simulink model "gm_PMLSM_FOC_FixedPoint"  (R2026b)
settings: Solver=FixedStepDiscrete  StopTime=0.0063  FixedStep=2e-08
undefined symbols (not defined in the file): Lookup, Ts_ACR
libraries: hdlmdlgenlib x38, simulink x8
(part 2 of 5)

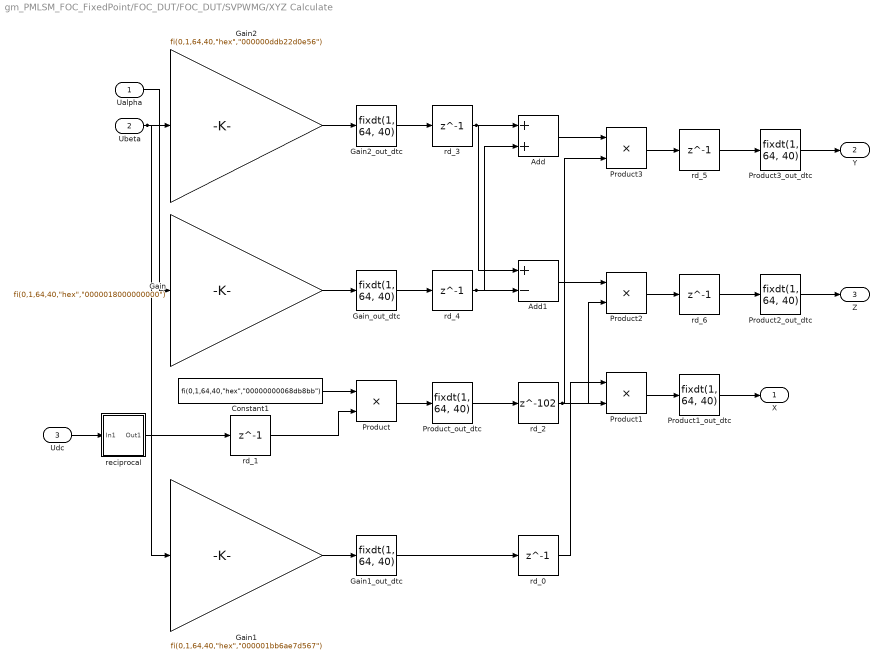
== system gm_PMLSM_FOC_FixedPoint/FOC_DUT/FOC_DUT/SVPWMG/XYZ Calculate ==
  Ualpha : Inport  OutDataTypeStr=fixdt(1, 64, 40)  PortDimensions=1  SampleTime=2e-08
  Ubeta : Inport  Port=2  OutDataTypeStr=fixdt(1, 64, 40)  PortDimensions=1  SampleTime=2e-08
  Udc : Inport  Port=3  OutDataTypeStr=fixdt(0, 32, 24)  PortDimensions=1  SampleTime=2e-08
  Add : Sum  OutDataTypeStr=fixdt(1, 64, 40)  AccumDataTypeStr=fixdt(1, 64, 40)  RndMeth=Convergent  SaturateOnIntegerOverflow=on  SampleTime=2e-08
  Add1 : Sum  Inputs=+-  OutDataTypeStr=fixdt(1, 64, 40)  AccumDataTypeStr=fixdt(1, 64, 40)  RndMeth=Convergent  SaturateOnIntegerOverflow=on  SampleTime=2e-08
  Constant1 : Constant  Value="fi(0,1,64,40,\"hex\",\"00000000068db8bb\")"  OutDataTypeStr=fixdt(1, 64, 40)  SampleTime=2e-08
  Gain : Gain  Gain="fi(0,1,64,40,\"hex\",\"0000018000000000\")"  ParamDataTypeStr=fixdt(1, 64, 40)  OutDataTypeStr=fixdt(1, 128, 80)  SampleTime=2e-08
  Gain1 : Gain  Gain="fi(0,1,64,40,\"hex\",\"000001bb6ae7d567\")"  ParamDataTypeStr=fixdt(1, 64, 40)  OutDataTypeStr=fixdt(1, 128, 80)  SampleTime=2e-08
  Gain1_out_dtc : DataTypeConversion  OutDataTypeStr=fixdt(1, 64, 40)  RndMeth=Convergent  SampleTime=2e-08
  Gain2 : Gain  Gain="fi(0,1,64,40,\"hex\",\"000000ddb22d0e56\")"  ParamDataTypeStr=fixdt(1, 64, 40)  OutDataTypeStr=fixdt(1, 128, 80)  SampleTime=2e-08
  Gain2_out_dtc : DataTypeConversion  OutDataTypeStr=fixdt(1, 64, 40)  RndMeth=Convergent  SampleTime=2e-08
  Gain_out_dtc : DataTypeConversion  OutDataTypeStr=fixdt(1, 64, 40)  RndMeth=Convergent  SampleTime=2e-08
  Product{,1..3} (4 alike) : Product  Inputs=**  OutDataTypeStr=fixdt(1, 128, 80)  SampleTime=2e-08
  Product1_out_dtc : DataTypeConversion  OutDataTypeStr=fixdt(1, 64, 40)  RndMeth=Convergent  SampleTime=2e-08
  Product2_out_dtc : DataTypeConversion  OutDataTypeStr=fixdt(1, 64, 40)  RndMeth=Convergent  SampleTime=2e-08
  Product3_out_dtc : DataTypeConversion  OutDataTypeStr=fixdt(1, 64, 40)  RndMeth=Convergent  SampleTime=2e-08
  Product_out_dtc : DataTypeConversion  OutDataTypeStr=fixdt(1, 64, 40)  RndMeth=Convergent  SampleTime=2e-08
  rd_{0..1,3..6} (6 alike) : Delay  DelayLength=1  InitialCondition=0  SampleTime=2e-08
  rd_2 : Delay  DelayLength=102  InitialCondition=0  SampleTime=2e-08
  reciprocal : Subsystem
  X : Outport  OutDataTypeStr=fixdt(1, 64, 40)  PortDimensions=1  SampleTime=2e-08
  Y : Outport  Port=2  OutDataTypeStr=fixdt(1, 64, 40)  PortDimensions=1  SampleTime=2e-08
  Z : Outport  Port=3  OutDataTypeStr=fixdt(1, 64, 40)  PortDimensions=1  SampleTime=2e-08
  wires:
  rd_3/1 -> Add1/1, Add/1
  Udc/1 -> reciprocal/1(In1)
  Ualpha/1 -> Gain/1
  Ubeta/1 -> Gain2/1, Gain1/1
  Gain2/1 -> Gain2_out_dtc/1
  Gain1_out_dtc/1 -> rd_0/1
  reciprocal/1(Out1) -> rd_1/1
  rd_1/1 -> Product/2
  Gain/1 -> Gain_out_dtc/1
  Constant1/1 -> Product/1
  Gain1/1 -> Gain1_out_dtc/1
  Gain2_out_dtc/1 -> rd_3/1
  Gain_out_dtc/1 -> rd_4/1
  Product/1 -> Product_out_dtc/1
  rd_4/1 -> Add1/2, Add/2
  Product_out_dtc/1 -> rd_2/1
  Add/1 -> Product3/1
  Product1/1 -> Product1_out_dtc/1
  Add1/1 -> Product2/1
  rd_2/1 -> Product1/2, Product3/2, Product2/2
  rd_0/1 -> Product1/1
  Product3/1 -> rd_5/1
  Product2/1 -> rd_6/1
  rd_5/1 -> Product3_out_dtc/1
  Product1_out_dtc/1 -> X/1
  rd_6/1 -> Product2_out_dtc/1
  Product3_out_dtc/1 -> Y/1
  Product2_out_dtc/1 -> Z/1

== system gm_PMLSM_FOC_FixedPoint/FOC_DUT/FOC_DUT/dq_voltage_limiter/Divide ==
  In1 : Inport
  In2 : Inport  Port=2
  Divide : Product  Inputs=*/  OutDataTypeStr=FOC_Fixed_Config.Types.DivideWide  RndMeth=Convergent  SaturateOnIntegerOverflow=on
  Divide_pd1 : Delay  DelayLength=109
  Out1 : Outport
  wires:
  Divide_pd1/1 -> Out1/1
  In1/1 -> Divide/1
  In2/1 -> Divide/2
  Divide/1 -> Divide_pd1/1

== system gm_PMLSM_FOC_FixedPoint/FOC_DUT/FOC_DUT/dq_voltage_limiter/Sqrt ==
  In1 : Inport
  Delay2 : Delay  DelayLength=56
  Sqrt : Sqrt  OutDataTypeStr=FOC_Fixed_Config.Types.Work
  Out1 : Outport
  wires:
  In1/1 -> Sqrt/1
  Sqrt/1 -> Delay2/1
  Delay2/1 -> Out1/1

== system gm_PMLSM_FOC_FixedPoint/FOC_DUT/FOC_DUT/InversePark/Variant/mcb ==
  A : Inport  OutDataTypeStr=fixdt(1, 64, 40)  PortDimensions=1  SampleTime=2e-08
  B : Inport  Port=2  OutDataTypeStr=fixdt(1, 64, 40)  PortDimensions=1  SampleTime=2e-08
  C : Inport  Port=3  OutDataTypeStr=fixdt(1, 40, 32)  PortDimensions=1  SampleTime=0.0001
  Inverse Park Transform : Subsystem  mask(Inverse Park Transform){PhaseInput=Two inputs, AxisAlignment=D-axis, ThetaInput=Sine and Cosine electrical position, AngleInput=Per-unit, N_points=1024}
      mask prompts: PhaseInput "mcb:CtrlLib:InvPPrmInp"; AxisAlignment "mcb:CtrlLib:InvPBlkPrmAlign"; ThetaInput "mcb:CtrlLib:InvPPrmTheta"; AngleInput "shared_mcbeeblks:mcbeeblks:InvPThetaUnits"; N_points "mcb:CtrlLib:SineBlkPrmLUTSize"
      mask help: mcb:CtrlLib:InvPBlkDlgDes
      mask init:
      | AngleInput = 2;
      | AxisAlignment = 'D-axis';
      | N_points = 1024;
      | PhaseInput = 1;
      | ThetaInput = 1;
      | dlgSett = struct('Offset', 0);
      mask Help: eval('mcb_helpview(''inverseparktransform'')')
      mask TypeOptions PhaseInput: shared_mcbeeblks:mcbeeblks:InvPPopTwo | shared_mcbeeblks:mcbeeblks:InvPPopThree
      mask TypeOptions AxisAlignment: D-axis | Q-axis
      mask TypeOptions ThetaInput: shared_mcbeeblks:mcbeeblks:InvPPopSinCos
      mask TypeOptions AngleInput: shared_mcbeeblks:mcbeeblks:InvPPopRadUnit | shared_mcbeeblks:mcbeeblks:InvPPopPUUnit | shared_mcbeeblks:mcbeeblks:InvPPopDegUnit
      mask Display:
      | port_label('input', 1, 'd', 'texmode', 'on');
      | port_label('input', 2, 'q', 'texmode', 'on');
      | port_label('input', 3, 'sin\theta_e', 'texmode', 'on');
      | port_label('input', 4, 'cos\theta_e', 'texmode', 'on');
      | port_label('output', 1, '\alpha', 'texmode', 'on');
      | port_label('output', 2, '\beta', 'texmode', 'on');
      | fprintf('Inverse Park\nTransform')
  sinecos : Subsystem  mask(SinCos Embedded Optimized){OptforProc=off, OptLevelPop=Disabled, ApproximationMethod='None', UserApproxMethod=Lookup, ApproxStatus=Lookup, ThetaDataType=single, CopyThetaDataType=single, InterpMethod='Linear point-slope', NumberOfDataPoints=16, NumberOfIterations=11, RemoveProtectionAgainstOutOfRangeInput='off', TableDataTypeStr='Inherit: Inherit via input', AngleInput='Radians', CopyAngleInput=Radians, N_points=N_points, CopyN_points=1024, Datatype='Inherit: Same as input', CopyTableDatatype=Inherit: Same as input, DatatypeInput='Inherit from input', IsPrevStrictOpt=0, IsPrevLUTForced=0}
      mask prompts: OptforProc "shared_mcbpccmath:SinCosLib:SineBlkOptimizeChkBox"; OptLevelPop "shared_mcbpccmath:SinCosLib:SineBlkOptimizePopMenu"; ApproximationMethod "Simulink:blkprm_prompts:ApproximationMethod"; UserApproxMethod "Simulink:blkprm_prompts:ApproximationMethod"; ApproxStatus "Simulink:blkprm_prompts:ApproximationMethod"; ThetaDataType "shared_mcbpccmath:SinCosLib:SineBlkPrmThetatype"; CopyThetaDataType "shared_mcbpccmath:SinCosLib:SineBlkPrmThetatype"; InterpMethod "Simulink:blkprm_prompts:InterpndInterpMethod"; NumberOfDataPoints "SimulinkBlocks:dialog:NumberOfDataPoints"; NumberOfIterations "SimulinkBlocks:dialog:NumberOfIterations"; RemoveProtectionAgainstOutOfRangeInput "Simulink:blkprm_prompts:TrigRemoveProtectionAgainstOutOfRangeInput"; TableDataTypeStr "Simulink:blkprm_prompts:TABLE_UNIFIEDDATATYPE"; AngleInput "shared_mcbpccmath:SinCosLib:SineBlkPrmUnits"; CopyAngleInput "shared_mcbpccmath:SinCosLib:SineBlkPrmUnits"; N_points "shared_mcbpccmath:SinCosLib:SineBlkPrmLUTSize"; CopyN_points "shared_mcbpccmath:SinCosLib:SineBlkPrmLUTSize"; Datatype "shared_mcbpccmath:SinCosLib:SineBlkPrmDatatype"; CopyTableDatatype "shared_mcbpccmath:SinCosLib:SineBlkPrmDatatype"; DatatypeInput "shared_mcbpccmath:SinCosLib:SineBlkPrmDatatypeInput"; IsPrevStrictOpt "Prev Strict Opt"; IsPrevLUTForced "Prev LUT Forced"
      mask help: mcb:CtrlLib:SineBlkDlgDes
      mask init:
      | AngleInput = 2;
      | ApproxStatus = [];
      | ApproximationMethod = 'None';
      | CopyAngleInput = 2;
      | CopyN_points = 1024;
      | CopyTableDatatype = 'Inherit: Same as input';
      | CopyThetaDataType = 'single';
      | Datatype = 'Inherit: Same as input';
      | DatatypeInput = 1;
      | InterpMethod = 'Linear point-slope';
      | IsPrevLUTForced = 0;
      | IsPrevStrictOpt = 0;
      | N_points = 1024;
      | NumberOfDataPoints = 16;
      | NumberOfIterations = 11;
      | OptLevelPop = 1;
      | OptforProc = 0;
      | RemoveProtectionAgainstOutOfRangeInput = 'off';
      | TableDataTypeStr = 'Inherit: Inherit via input';
      | ThetaDataType = 'single';
      | UserApproxMethod = 2;
      mask Help: eval('mcb_helpview(''sinecosinelookup'')')
      mask TypeOptions OptLevelPop: shared_mcbpccmath:SinCosLib:OptDisablePop | shared_mcbpccmath:SinCosLib:OptThetaOptimizationPop | shared_mcbpccmath:SinCosLib:OptStrictOptimizationPop
      mask Callback OptLevelPop: mcbpccmath.internal.SinCosMaskCb('maskInitFcn',gcbh);
      mask TypeOptions UserApproxMethod: shared_mcbpccmath:SinCosLib:SineApproxNone | shared_mcbpccmath:SinCosLib:SineApproxLookup | shared_mcbpccmath:SinCosLib:SineApproxCORDIC
      mask Callback UserApproxMethod: mcbpccmath.internal.SinCosMaskCb('maskInitFcn',gcbh);
      mask Callback ThetaDataType:
      | mcbpccmath.internal.SinCosMaskCb('updateCopyVar',gcbh,'ThetaDataType');
      | mcbpccmath.internal.SinCosMaskCb('maskInitFcn',gcbh);
      mask Callback AngleInput:
      | mcbpccmath.internal.SinCosMaskCb('updateCopyVar',gcbh,'AngleInput');
      | mcbpccmath.internal.SinCosMaskCb('maskInitFcn',gcbh);
      mask TypeOptions CopyAngleInput: shared_mcbpccmath:SinCosLib:SinePopPUUnit | shared_mcbpccmath:SinCosLib:SinePopRadUnit | shared_mcbpccmath:SinCosLib:SinePopDegUnit
      mask Callback N_points: mcbpccmath.internal.SinCosMaskCb('updateCopyVar',gcbh,'N_points');
      mask Callback Datatype: mcbpccmath.internal.SinCosMaskCb('updateCopyVar',gcbh,'Datatype');
      mask Display: mcbpccmath.internal.drawIcons('Sin-Cos',2);
  O1 : Outport  OutDataTypeStr=fixdt(1, 64, 40)  PortDimensions=1  SampleTime=2e-08
  O2 : Outport  Port=2  OutDataTypeStr=fixdt(1, 64, 40)  PortDimensions=1  SampleTime=2e-08
  wires:
  C/1 -> sinecos/1(Theta)
  A/1 -> Inverse Park Transform/1(Ds)
  Inverse Park Transform/2(Beta) -> O2/1
  B/1 -> Inverse Park Transform/2(Qs)
  sinecos/1(sin) -> Inverse Park Transform/3(Sin)
  sinecos/2(cos) -> Inverse Park Transform/4(Cos)
  Inverse Park Transform/1(Alpha) -> O1/1

== system gm_PMLSM_FOC_FixedPoint/FOC_DUT/FOC_DUT/Park/Variant/mcb ==
  A : Inport  OutDataTypeStr=fixdt(1, 64, 40)  PortDimensions=1  SampleTime=0.0001
  B : Inport  Port=2  OutDataTypeStr=fixdt(1, 64, 40)  PortDimensions=1  SampleTime=0.0001
  C : Inport  Port=3  OutDataTypeStr=fixdt(1, 40, 32)  PortDimensions=1  SampleTime=0.0001
  Park Transform : Subsystem  mask(Park Transform){PhaseInput=Two inputs, AxisAlignment=D-axis, ThetaInput=Sine and Cosine electrical position, AngleInput=Per-unit, N_points=1024}
      mask prompts: PhaseInput "mcb:CtrlLib:ParkPrmInp"; AxisAlignment "mcb:CtrlLib:ParkBlkPrmAlign"; ThetaInput "mcb:CtrlLib:ParkPrmTheta"; AngleInput "shared_mcbeeblks:mcbeeblks:ParkPrmThetaUnits"; N_points "mcb:CtrlLib:SineBlkPrmLUTSize"
      mask help: mcb:CtrlLib:ParkBlkDlgDes
      mask init:
      | AngleInput = 2;
      | AxisAlignment = 'D-axis';
      | N_points = 1024;
      | PhaseInput = 1;
      | ThetaInput = 1;
      | dlgSett = struct('Offset', 0);
      mask Help: eval('mcb_helpview(''parktransform'')')
      mask TypeOptions PhaseInput: shared_mcbeeblks:mcbeeblks:ParkPopTwo | shared_mcbeeblks:mcbeeblks:ParkPopThree
      mask TypeOptions AxisAlignment: D-axis | Q-axis
      mask TypeOptions ThetaInput: shared_mcbeeblks:mcbeeblks:ParkPopSinCos
      mask TypeOptions AngleInput: shared_mcbeeblks:mcbeeblks:ParkPopRadUnit | shared_mcbeeblks:mcbeeblks:ParkPopPUUnit | shared_mcbeeblks:mcbeeblks:ParkPopDegUnit
      mask Display:
      | port_label('input', 1, '\alpha', 'texmode', 'on');
      | port_label('input', 2, '\beta', 'texmode', 'on');
      | port_label('input', 3, 'sin\theta_e', 'texmode', 'on');
      | port_label('input', 4, 'cos\theta_e', 'texmode', 'on');
      | port_label('output', 1, 'd', 'texmode', 'on');
      | port_label('output', 2, 'q', 'texmode', 'on');
      | fprintf('Park\nTransform')
  sinecos : Subsystem  mask(SinCos Embedded Optimized){OptforProc=off, OptLevelPop=Disabled, ApproximationMethod='None', UserApproxMethod=Lookup, ApproxStatus=Lookup, ThetaDataType=single, CopyThetaDataType=single, InterpMethod='Linear point-slope', NumberOfDataPoints=16, NumberOfIterations=11, RemoveProtectionAgainstOutOfRangeInput='off', TableDataTypeStr='Inherit: Inherit via input', AngleInput='Radians', CopyAngleInput=Radians, N_points=N_points, CopyN_points=1024, Datatype='Inherit: Same as input', CopyTableDatatype=Inherit: Same as input, DatatypeInput='Inherit from input', IsPrevStrictOpt=0, IsPrevLUTForced=0}
      mask prompts: OptforProc "shared_mcbpccmath:SinCosLib:SineBlkOptimizeChkBox"; OptLevelPop "shared_mcbpccmath:SinCosLib:SineBlkOptimizePopMenu"; ApproximationMethod "Simulink:blkprm_prompts:ApproximationMethod"; UserApproxMethod "Simulink:blkprm_prompts:ApproximationMethod"; ApproxStatus "Simulink:blkprm_prompts:ApproximationMethod"; ThetaDataType "shared_mcbpccmath:SinCosLib:SineBlkPrmThetatype"; CopyThetaDataType "shared_mcbpccmath:SinCosLib:SineBlkPrmThetatype"; InterpMethod "Simulink:blkprm_prompts:InterpndInterpMethod"; NumberOfDataPoints "SimulinkBlocks:dialog:NumberOfDataPoints"; NumberOfIterations "SimulinkBlocks:dialog:NumberOfIterations"; RemoveProtectionAgainstOutOfRangeInput "Simulink:blkprm_prompts:TrigRemoveProtectionAgainstOutOfRangeInput"; TableDataTypeStr "Simulink:blkprm_prompts:TABLE_UNIFIEDDATATYPE"; AngleInput "shared_mcbpccmath:SinCosLib:SineBlkPrmUnits"; CopyAngleInput "shared_mcbpccmath:SinCosLib:SineBlkPrmUnits"; N_points "shared_mcbpccmath:SinCosLib:SineBlkPrmLUTSize"; CopyN_points "shared_mcbpccmath:SinCosLib:SineBlkPrmLUTSize"; Datatype "shared_mcbpccmath:SinCosLib:SineBlkPrmDatatype"; CopyTableDatatype "shared_mcbpccmath:SinCosLib:SineBlkPrmDatatype"; DatatypeInput "shared_mcbpccmath:SinCosLib:SineBlkPrmDatatypeInput"; IsPrevStrictOpt "Prev Strict Opt"; IsPrevLUTForced "Prev LUT Forced"
      mask help: mcb:CtrlLib:SineBlkDlgDes
      mask init: same as gm_PMLSM_FOC_FixedPoint/FOC_DUT/FOC_DUT/InversePark/Variant/mcb/sinecos
      mask Help: eval('mcb_helpview(''sinecosinelookup'')')
      mask TypeOptions OptLevelPop: shared_mcbpccmath:SinCosLib:OptDisablePop | shared_mcbpccmath:SinCosLib:OptThetaOptimizationPop | shared_mcbpccmath:SinCosLib:OptStrictOptimizationPop
      mask Callback OptLevelPop: mcbpccmath.internal.SinCosMaskCb('maskInitFcn',gcbh);
      mask TypeOptions UserApproxMethod: shared_mcbpccmath:SinCosLib:SineApproxNone | shared_mcbpccmath:SinCosLib:SineApproxLookup | shared_mcbpccmath:SinCosLib:SineApproxCORDIC
      mask Callback UserApproxMethod: mcbpccmath.internal.SinCosMaskCb('maskInitFcn',gcbh);
      mask Callback ThetaDataType:
      | mcbpccmath.internal.SinCosMaskCb('updateCopyVar',gcbh,'ThetaDataType');
      | mcbpccmath.internal.SinCosMaskCb('maskInitFcn',gcbh);
      mask Callback AngleInput:
      | mcbpccmath.internal.SinCosMaskCb('updateCopyVar',gcbh,'AngleInput');
      | mcbpccmath.internal.SinCosMaskCb('maskInitFcn',gcbh);
      mask TypeOptions CopyAngleInput: shared_mcbpccmath:SinCosLib:SinePopPUUnit | shared_mcbpccmath:SinCosLib:SinePopRadUnit | shared_mcbpccmath:SinCosLib:SinePopDegUnit
      mask Callback N_points: mcbpccmath.internal.SinCosMaskCb('updateCopyVar',gcbh,'N_points');
      mask Callback Datatype: mcbpccmath.internal.SinCosMaskCb('updateCopyVar',gcbh,'Datatype');
      mask Display: mcbpccmath.internal.drawIcons('Sin-Cos',2);
  O1 : Outport  OutDataTypeStr=fixdt(1, 64, 40)  PortDimensions=1  SampleTime=0.0001
  O2 : Outport  Port=2  OutDataTypeStr=fixdt(1, 64, 40)  PortDimensions=1  SampleTime=0.0001
  wires:
  Park Transform/1(Ds) -> O1/1
  sinecos/2(cos) -> Park Transform/4(Cos)
  C/1 -> sinecos/1(Theta)
  A/1 -> Park Transform/1(Alpha)
  B/1 -> Park Transform/2(Beta)
  sinecos/1(sin) -> Park Transform/3(Sin)
  Park Transform/2(Qs) -> O2/1

== system gm_PMLSM_FOC_FixedPoint/FOC_DUT/FOC_DUT/SVPWMG/Duty Calculate/Fcn ==
  Vector : Inport  OutDataTypeStr=fixdt(1, 64, 40)  PortDimensions=[3]  SampleTime=2e-08
  Combination_stage2 : Sum  Inputs=+-  OutDataTypeStr=fixdt(1, 64, 40)  AccumDataTypeStr=fixdt(1, 64, 40)  RndMeth=Convergent  SaturateOnIntegerOverflow=on  SampleTime=2e-08
  Combination_stage3 : Sum  Inputs=+-  OutDataTypeStr=fixdt(1, 64, 40)  AccumDataTypeStr=fixdt(1, 64, 40)  RndMeth=Convergent  SaturateOnIntegerOverflow=on  SampleTime=2e-08
  Quarter : Gain  Gain="fi(0,1,64,40,\"hex\",\"0000004000000000\")"  ParamDataTypeStr=fixdt(1, 64, 40)  OutDataTypeStr=fixdt(1, 64, 40)  RndMeth=Convergent  SaturateOnIntegerOverflow=on  SampleTime=2e-08
  rd_0 : Delay  DelayLength=1  InitialCondition=0  SampleTime=2e-08
  t : Demux  Outputs=3
  Value : Outport  OutDataTypeStr=fixdt(1, 64, 40)  PortDimensions=1  SampleTime=2e-08
  wires:
  Vector/1 -> t/1
  t/1 -> Combination_stage2/2
  Combination_stage2/1 -> Combination_stage3/1
  t/2 -> Combination_stage3/2
  t/3 -> Combination_stage2/1
  Quarter/1 -> Value/1
  rd_0/1 -> Quarter/1
  Combination_stage3/1 -> rd_0/1

== system gm_PMLSM_FOC_FixedPoint/FOC_DUT/FOC_DUT/SVPWMG/Duty Calculate/Fcn1 ==
  Vector : Inport  OutDataTypeStr=fixdt(1, 64, 40)  PortDimensions=[3]  SampleTime=2e-08
  Combination_stage2 : Sum  OutDataTypeStr=fixdt(1, 64, 40)  AccumDataTypeStr=fixdt(1, 64, 40)  RndMeth=Convergent  SaturateOnIntegerOverflow=on  SampleTime=2e-08
  Combination_stage3 : Sum  Inputs=+-  OutDataTypeStr=fixdt(1, 64, 40)  AccumDataTypeStr=fixdt(1, 64, 40)  RndMeth=Convergent  SaturateOnIntegerOverflow=on  SampleTime=2e-08
  Quarter : Gain  Gain="fi(0,1,64,40,\"hex\",\"0000004000000000\")"  ParamDataTypeStr=fixdt(1, 64, 40)  OutDataTypeStr=fixdt(1, 64, 40)  RndMeth=Convergent  SaturateOnIntegerOverflow=on  SampleTime=2e-08
  rd_0 : Delay  DelayLength=1  InitialCondition=0  SampleTime=2e-08
  t : Demux  Outputs=3
  Value : Outport  OutDataTypeStr=fixdt(1, 64, 40)  PortDimensions=1  SampleTime=2e-08
  wires:
  Vector/1 -> t/1
  t/1 -> Combination_stage2/2
  Combination_stage2/1 -> Combination_stage3/1
  t/2 -> Combination_stage3/2
  t/3 -> Combination_stage2/1
  Quarter/1 -> Value/1
  rd_0/1 -> Quarter/1
  Combination_stage3/1 -> rd_0/1

== system gm_PMLSM_FOC_FixedPoint/FOC_DUT/FOC_DUT/SVPWMG/Duty Calculate/Fcn2 ==
  Vector : Inport  OutDataTypeStr=fixdt(1, 64, 40)  PortDimensions=[3]  SampleTime=2e-08
  Combination_stage2 : Sum  OutDataTypeStr=fixdt(1, 64, 40)  AccumDataTypeStr=fixdt(1, 64, 40)  RndMeth=Convergent  SaturateOnIntegerOverflow=on  SampleTime=2e-08
  Combination_stage3 : Sum  OutDataTypeStr=fixdt(1, 64, 40)  AccumDataTypeStr=fixdt(1, 64, 40)  RndMeth=Convergent  SaturateOnIntegerOverflow=on  SampleTime=2e-08
  Quarter : Gain  Gain="fi(0,1,64,40,\"hex\",\"0000004000000000\")"  ParamDataTypeStr=fixdt(1, 64, 40)  OutDataTypeStr=fixdt(1, 64, 40)  RndMeth=Convergent  SaturateOnIntegerOverflow=on  SampleTime=2e-08
  rd_0 : Delay  DelayLength=1  InitialCondition=0  SampleTime=2e-08
  t : Demux  Outputs=3
  Value : Outport  OutDataTypeStr=fixdt(1, 64, 40)  PortDimensions=1  SampleTime=2e-08
  wires:
  Vector/1 -> t/1
  t/1 -> Combination_stage3/2
  Combination_stage2/1 -> Combination_stage3/1
  t/2 -> Combination_stage2/2
  t/3 -> Combination_stage2/1
  Quarter/1 -> Value/1
  rd_0/1 -> Quarter/1
  Combination_stage3/1 -> rd_0/1

== system gm_PMLSM_FOC_FixedPoint/FOC_DUT/FOC_DUT/SVPWMG/Sector Caculate/B0 ==
  Vector : Inport  OutDataTypeStr=fixdt(1, 64, 40)  PortDimensions=[2]  SampleTime=2e-08
  Vector_0_term0 : Terminator
  t : Demux  Outputs=2
  Value : Outport  OutDataTypeStr=fixdt(1, 64, 40)  PortDimensions=1  SampleTime=2e-08
  wires:
  t/2 -> Value/1
  Vector/1 -> t/1
  t/1 -> Vector_0_term0/1

== system gm_PMLSM_FOC_FixedPoint/FOC_DUT/FOC_DUT/SVPWMG/Sector Caculate/B1 ==
  Vector : Inport  OutDataTypeStr=fixdt(1, 64, 40)  PortDimensions=[2]  SampleTime=2e-08
  Alpha0866 : Gain  Gain="fi(0,1,64,40,\"hex\",\"000000ddb22d0e56\")"  ParamDataTypeStr=fixdt(1, 64, 40)  OutDataTypeStr=fixdt(1, 128, 80)  SampleTime=2e-08
  Alpha0866_out_dtc : DataTypeConversion  OutDataTypeStr=fixdt(1, 64, 40)  RndMeth=Convergent  SampleTime=2e-08
  Beta05 : Gain  Gain="fi(0,1,64,40,\"hex\",\"0000008000000000\")"  ParamDataTypeStr=fixdt(1, 64, 40)  OutDataTypeStr=fixdt(1, 64, 40)  RndMeth=Convergent  SaturateOnIntegerOverflow=on  SampleTime=2e-08
  Projection : Sum  Inputs=+-  OutDataTypeStr=fixdt(1, 64, 40)  AccumDataTypeStr=fixdt(1, 64, 40)  RndMeth=Convergent  SaturateOnIntegerOverflow=on  SampleTime=2e-08
  rd_0 : Delay  DelayLength=1  InitialCondition=0  SampleTime=2e-08
  rd_1 : Delay  DelayLength=1  InitialCondition=0  SampleTime=2e-08
  t : Demux  Outputs=2
  Value : Outport  OutDataTypeStr=fixdt(1, 64, 40)  PortDimensions=1  SampleTime=2e-08
  wires:
  Alpha0866_out_dtc/1 -> rd_0/1
  t/1 -> Alpha0866/1
  Vector/1 -> t/1
  t/2 -> Beta05/1
  Alpha0866/1 -> Alpha0866_out_dtc/1
  Beta05/1 -> rd_1/1
  rd_0/1 -> Projection/1
  rd_1/1 -> Projection/2
  Projection/1 -> Value/1

== system gm_PMLSM_FOC_FixedPoint/FOC_DUT/FOC_DUT/SVPWMG/Sector Caculate/B2 ==
  Vector : Inport  OutDataTypeStr=fixdt(1, 64, 40)  PortDimensions=[2]  SampleTime=2e-08
  Alpha0866 : Gain  Gain="fi(0,1,64,40,\"hex\",\"000000ddb22d0e56\")"  ParamDataTypeStr=fixdt(1, 64, 40)  OutDataTypeStr=fixdt(1, 128, 80)  SampleTime=2e-08
  Alpha0866_out_dtc : DataTypeConversion  OutDataTypeStr=fixdt(1, 64, 40)  RndMeth=Convergent  SampleTime=2e-08
  Beta05 : Gain  Gain="fi(0,1,64,40,\"hex\",\"0000008000000000\")"  ParamDataTypeStr=fixdt(1, 64, 40)  OutDataTypeStr=fixdt(1, 64, 40)  RndMeth=Convergent  SaturateOnIntegerOverflow=on  SampleTime=2e-08
  Projection : Sum  Inputs=--  OutDataTypeStr=fixdt(1, 64, 40)  AccumDataTypeStr=fixdt(1, 64, 40)  RndMeth=Convergent  SaturateOnIntegerOverflow=on  SampleTime=2e-08
  rd_0 : Delay  DelayLength=1  InitialCondition=0  SampleTime=2e-08
  rd_1 : Delay  DelayLength=1  InitialCondition=0  SampleTime=2e-08
  t : Demux  Outputs=2
  Value : Outport  OutDataTypeStr=fixdt(1, 64, 40)  PortDimensions=1  SampleTime=2e-08
  wires:
  t/2 -> Beta05/1
  Vector/1 -> t/1
  Alpha0866_out_dtc/1 -> rd_0/1
  t/1 -> Alpha0866/1
  Alpha0866/1 -> Alpha0866_out_dtc/1
  Beta05/1 -> rd_1/1
  rd_0/1 -> Projection/1
  rd_1/1 -> Projection/2
  Projection/1 -> Value/1

== system gm_PMLSM_FOC_FixedPoint/FOC_DUT/FOC_DUT/SVPWMG/Sector Caculate/N ==
  Vector : Inport  OutDataTypeStr=uint8  PortDimensions=[3]  SampleTime=2e-08
  Four : Gain  Gain="fi(0,0,8,0,\"hex\",\"04\")"  ParamDataTypeStr=fixdt(0, 8, 0)  OutDataTypeStr=uint8  RndMeth=Convergent  SaturateOnIntegerOverflow=on  SampleTime=2e-08
  SectorNumber_stage2 : Sum  OutDataTypeStr=uint8  AccumDataTypeStr=uint8  RndMeth=Convergent  SaturateOnIntegerOverflow=on  SampleTime=2e-08
  SectorNumber_stage3 : Sum  OutDataTypeStr=uint8  AccumDataTypeStr=uint8  RndMeth=Convergent  SaturateOnIntegerOverflow=on  SampleTime=2e-08
  Two : Gain  Gain="fi(0,0,8,0,\"hex\",\"02\")"  ParamDataTypeStr=fixdt(0, 8, 0)  OutDataTypeStr=uint8  RndMeth=Convergent  SaturateOnIntegerOverflow=on  SampleTime=2e-08
  rd_0 : Delay  DelayLength=1  InitialCondition=0  SampleTime=2e-08
  rd_1 : Delay  DelayLength=1  InitialCondition=0  SampleTime=2e-08
  rd_2 : Delay  DelayLength=1  InitialCondition=0  SampleTime=2e-08
  rd_3 : Delay  InitialCondition=0  SampleTime=2e-08
  t : Demux  Outputs=3
  Value : Outport  OutDataTypeStr=uint8  PortDimensions=1  SampleTime=2e-08
  wires:
  SectorNumber_stage3/1 -> Value/1
  Four/1 -> SectorNumber_stage2/1
  rd_0/1 -> Four/1
  t/3 -> rd_0/1
  Vector/1 -> t/1
  rd_1/1 -> Two/1
  t/1 -> rd_3/1
  t/2 -> rd_1/1
  Two/1 -> SectorNumber_stage2/2
  rd_3/1 -> SectorNumber_stage3/2
  SectorNumber_stage2/1 -> rd_2/1
  rd_2/1 -> SectorNumber_stage3/1

== system gm_PMLSM_FOC_FixedPoint/FOC_DUT/FOC_DUT/SVPWMG/T1T2 Calculate/Fcn ==
  Vector : Inport  OutDataTypeStr=fixdt(1, 64, 40)  PortDimensions=[3]  SampleTime=2e-08
  Combination_stage2 : Sum  Inputs=+-  OutDataTypeStr=fixdt(1, 64, 40)  AccumDataTypeStr=fixdt(1, 64, 40)  RndMeth=Convergent  SaturateOnIntegerOverflow=on  SampleTime=2e-08
  Combination_stage3 : Sum  Inputs=+-  OutDataTypeStr=fixdt(1, 64, 40)  AccumDataTypeStr=fixdt(1, 64, 40)  RndMeth=Convergent  SaturateOnIntegerOverflow=on  SampleTime=2e-08
  rd_0 : Delay  DelayLength=1  InitialCondition=0  SampleTime=2e-08
  rd_1 : Delay  DelayLength=1  InitialCondition=0  SampleTime=2e-08
  t : Demux  Outputs=3
  Value : Outport  OutDataTypeStr=fixdt(1, 64, 40)  PortDimensions=1  SampleTime=2e-08
  wires:
  t/3 -> Combination_stage2/1
  Vector/1 -> t/1
  rd_1/1 -> Combination_stage3/2
  t/1 -> rd_1/1
  Combination_stage2/1 -> rd_0/1
  t/2 -> Combination_stage2/2
  Combination_stage3/1 -> Value/1
  rd_0/1 -> Combination_stage3/1

== system gm_PMLSM_FOC_FixedPoint/FOC_DUT/FOC_DUT/SVPWMG/T1T2 Calculate/Fcn1 ==
  Vector : Inport  OutDataTypeStr=fixdt(1, 64, 40)  PortDimensions=[3]  SampleTime=2e-08
  Defined_Fallback : Constant  Value="fi(0,1,64,40,\"hex\",\"0000010000000000\")"  OutDataTypeStr=fixdt(1, 64, 40)  SampleTime=2e-08
  Defined_Quotient : Subsystem
  Denominator_Nonzero : simulink/Logic and Bit Operations/Compare To Constant  relop=~=  const=0  OutDataTypeStr=boolean
  Numerator : Product  Inputs=**  OutDataTypeStr=fixdt(1, 128, 80)  SampleTime=2e-08
  Numerator_out_dtc : DataTypeConversion  OutDataTypeStr=fixdt(1, 64, 40)  RndMeth=Convergent  SampleTime=2e-08
  Safe_Denominator : Switch  Criteria=u2 ~= 0  Threshold="fi(0,0,1,0,\"hex\",\"0\")"  OutDataTypeStr=fixdt(1, 64, 40)  RndMeth=Convergent  SampleTime=2e-08  InputSameDT=off
  Sum_Times : Sum  OutDataTypeStr=fixdt(1, 64, 40)  AccumDataTypeStr=fixdt(1, 64, 40)  RndMeth=Convergent  SaturateOnIntegerOverflow=on  SampleTime=2e-08
  default_value : Constant  Value=fi(1,1,64,40)  OutDataTypeStr=fixdt(1, 64, 40)  SampleTime=2e-08
  delayMatch : Delay  DelayLength=179  InitialCondition=0  SampleTime=2e-08
  rd_0 : Delay  DelayLength=1  InitialCondition=0  SampleTime=2e-08
  rd_1 : Delay  DelayLength=1  InitialCondition=0  SampleTime=2e-08
  select_signal : Constant  OutDataTypeStr=boolean  SampleTime=2e-08
  t : Demux  Outputs=3
  zero_protection : Switch  Criteria=u2 ~= 0  OutDataTypeStr=fixdt(1, 64, 40)  SampleTime=2e-08  SaturateOnIntegerOverflow=off  InputSameDT=off
  Value : Outport  OutDataTypeStr=fixdt(1, 64, 40)  PortDimensions=1  SampleTime=2e-08
  wires:
  t/3 -> Numerator/2
  Vector/1 -> t/1
  t/1 -> Sum_Times/1, Numerator/1
  rd_0/1 -> Numerator_out_dtc/1
  t/2 -> Sum_Times/2
  rd_1/1 -> Safe_Denominator/1, Denominator_Nonzero/1
  Numerator/1 -> rd_0/1
  Sum_Times/1 -> rd_1/1
  Denominator_Nonzero/1 -> Safe_Denominator/2
  Defined_Fallback/1 -> Safe_Denominator/3
  select_signal/1 -> delayMatch/1
  Safe_Denominator/1 -> zero_protection/1
  delayMatch/1 -> zero_protection/2
  default_value/1 -> zero_protection/3
  Numerator_out_dtc/1 -> Defined_Quotient/1(In1)
  Defined_Quotient/1(Out1) -> Value/1
  zero_protection/1 -> Defined_Quotient/2(In2)

== system gm_PMLSM_FOC_FixedPoint/FOC_DUT/FOC_DUT/SVPWMG/T1T2 Calculate/Fcn2 ==
  Vector : Inport  OutDataTypeStr=fixdt(1, 64, 40)  PortDimensions=[3]  SampleTime=2e-08
  Defined_Fallback : Constant  Value="fi(0,1,64,40,\"hex\",\"0000010000000000\")"  OutDataTypeStr=fixdt(1, 64, 40)  SampleTime=2e-08
  Defined_Quotient : Subsystem
  Denominator_Nonzero : simulink/Logic and Bit Operations/Compare To Constant  relop=~=  const=0  OutDataTypeStr=boolean
  Numerator : Product  Inputs=**  OutDataTypeStr=fixdt(1, 128, 80)  SampleTime=2e-08
  Numerator_out_dtc : DataTypeConversion  OutDataTypeStr=fixdt(1, 64, 40)  RndMeth=Convergent  SampleTime=2e-08
  Safe_Denominator : Switch  Criteria=u2 ~= 0  Threshold="fi(0,0,1,0,\"hex\",\"0\")"  OutDataTypeStr=fixdt(1, 64, 40)  RndMeth=Convergent  SampleTime=2e-08  InputSameDT=off
  Sum_Times : Sum  OutDataTypeStr=fixdt(1, 64, 40)  AccumDataTypeStr=fixdt(1, 64, 40)  RndMeth=Convergent  SaturateOnIntegerOverflow=on  SampleTime=2e-08
  default_value : Constant  Value=fi(1,1,64,40)  OutDataTypeStr=fixdt(1, 64, 40)  SampleTime=2e-08
  delayMatch : Delay  DelayLength=179  InitialCondition=0  SampleTime=2e-08
  rd_0 : Delay  DelayLength=1  InitialCondition=0  SampleTime=2e-08
  rd_1 : Delay  DelayLength=1  InitialCondition=0  SampleTime=2e-08
  select_signal : Constant  OutDataTypeStr=boolean  SampleTime=2e-08
  t : Demux  Outputs=3
  zero_protection : Switch  Criteria=u2 ~= 0  OutDataTypeStr=fixdt(1, 64, 40)  SampleTime=2e-08  SaturateOnIntegerOverflow=off  InputSameDT=off
  Value : Outport  OutDataTypeStr=fixdt(1, 64, 40)  PortDimensions=1  SampleTime=2e-08
  wires:
  Sum_Times/1 -> rd_1/1
  Vector/1 -> t/1
  t/3 -> Numerator/2
  Defined_Fallback/1 -> Safe_Denominator/3
  t/1 -> Sum_Times/1
  rd_0/1 -> Numerator_out_dtc/1
  t/2 -> Sum_Times/2, Numerator/1
  Numerator/1 -> rd_0/1
  rd_1/1 -> Safe_Denominator/1, Denominator_Nonzero/1
  delayMatch/1 -> zero_protection/2
  Denominator_Nonzero/1 -> Safe_Denominator/2
  select_signal/1 -> delayMatch/1
  Safe_Denominator/1 -> zero_protection/1
  default_value/1 -> zero_protection/3
  Numerator_out_dtc/1 -> Defined_Quotient/1(In1)
  zero_protection/1 -> Defined_Quotient/2(In2)
  Defined_Quotient/1(Out1) -> Value/1

== system gm_PMLSM_FOC_FixedPoint/FOC_DUT/FOC_DUT/SVPWMG/XYZ Calculate/reciprocal ==
  In1 : Inport
  reciprocal : Math  Operator=reciprocal  OutDataTypeStr=FOC_Fixed_Config.Types.Work  RndMeth=Convergent
  reciprocal_pd1 : Delay  DelayLength=71
  Out1 : Outport
  wires:
  In1/1 -> reciprocal/1
  reciprocal/1 -> reciprocal_pd1/1
  reciprocal_pd1/1 -> Out1/1

== system gm_PMLSM_FOC_FixedPoint/FOC_DUT/FOC_DUT/InversePark/Variant/mcb/Inverse Park Transform ==
  Ds : Inport  OutDataTypeStr=fixdt(1,64,40,'DataTypeOverride', 'Off')  PortDimensions=1  SampleTime=2e-08
  Qs : Inport  Port=2  OutDataTypeStr=fixdt(1,64,40,'DataTypeOverride', 'Off')  PortDimensions=1  SampleTime=2e-08
  Sin : Inport  Port=3  OutDataTypeStr=fixdt(1,40,32,'DataTypeOverride', 'Off')  PortDimensions=1  SampleTime=2e-08
  Cos : Inport  Port=4  OutDataTypeStr=fixdt(1,40,32,'DataTypeOverride', 'Off')  PortDimensions=1  SampleTime=2e-08
  Select : Subsystem
  Alpha : Outport  OutDataTypeStr=fixdt(1, 64, 40)  PortDimensions=1  SampleTime=2e-08  VectorParamsAs1DForOutWhenUnconnected=off
  Beta : Outport  Port=2  OutDataTypeStr=fixdt(1, 64, 40)  PortDimensions=1  SampleTime=2e-08
  wires:
  Ds/1 -> Select/1(D)
  Qs/1 -> Select/2(Q)
  Select/1(AlphaO) -> Alpha/1
  Sin/1 -> Select/3(Sin)
  Cos/1 -> Select/4(Cos)
  Select/2(BetaO) -> Beta/1

== system gm_PMLSM_FOC_FixedPoint/FOC_DUT/FOC_DUT/InversePark/Variant/mcb/sinecos ==
  note: For TI proc with fixed-point datatype
  Theta : Inport  OutDataTypeStr=fixdt(1,40,32,'DataTypeOverride', 'Off')  PortDimensions=1  SampleTime=0.0001
  Sine-Cosine Lookup : Subsystem  mask(Sine-Cosine Lookup){AngleInput=Radians, N_points=1024, DatatypeInput=Inherit from input, Datatype=Inherit: Same as input}
      mask prompts: AngleInput "shared_mcbpccmath:SinCosLib:SineBlkPrmUnits"; N_points "shared_mcbpccmath:SinCosLib:SineBlkPrmLUTSize"; DatatypeInput "shared_mcbpccmath:SinCosLib:SineBlkPrmDatatypeInput"; Datatype "shared_mcbpccmath:SinCosLib:SineBlkPrmDatatype"
      mask help: mcb:CtrlLib:SineBlkDlgDes
      mask init:
      | AngleInput = 2;
      | Datatype = 'Inherit: Same as input';
      | DatatypeInput = 1;
      | N_points = 1024;
      mask Help: eval('mcb_helpview(''sinecosinelookup'')')
      mask TypeOptions AngleInput: shared_mcbpccmath:SinCosLib:SinePopPUUnit | shared_mcbpccmath:SinCosLib:SinePopRadUnit | shared_mcbpccmath:SinCosLib:SinePopDegUnit
      mask TypeOptions DatatypeInput: shared_mcbpccmath:SinCosLib:SineBlkPopIn | shared_mcbpccmath:SinCosLib:SineBlkPopDlg
      mask Callback DatatypeInput:
      | InputFormat = get_param(gcbh,'DatatypeInput');
      | Mask = Simulink.Mask.get(gcbh);
      | Datatype = Mask.getParameter('Datatype');
      | if(strcmp(InputFormat,'Inherit from input'))
      |     Datatype.Visible = 'off';
      | else
      |     Datatype.Visible = 'on';
      | end
      mask Display: mcbpccmath.internal.drawIcons('Sin-Cos',1);
  sin : Outport  OutDataTypeStr=fixdt(1, 40, 32)  PortDimensions=1  SampleTime=2e-08
  cos : Outport  Port=2  OutDataTypeStr=fixdt(1, 40, 32)  PortDimensions=1  SampleTime=2e-08
  wires:
  Theta/1 -> Sine-Cosine Lookup/1(Theta)
  Sine-Cosine Lookup/1(sin) -> sin/1
  Sine-Cosine Lookup/2(cos) -> cos/1

== system gm_PMLSM_FOC_FixedPoint/FOC_DUT/FOC_DUT/Park/Variant/mcb/Park Transform ==
  Alpha : Inport  OutDataTypeStr=fixdt(1,64,40,'DataTypeOverride', 'Off')  PortDimensions=1  SampleTime=0.0001
  Beta : Inport  Port=2  OutDataTypeStr=fixdt(1,64,40,'DataTypeOverride', 'Off')  PortDimensions=1  SampleTime=0.0001
  Sin : Inport  Port=3  OutDataTypeStr=fixdt(1,40,32,'DataTypeOverride', 'Off')  PortDimensions=1  SampleTime=0.0001
  Cos : Inport  Port=4  OutDataTypeStr=fixdt(1,40,32,'DataTypeOverride', 'Off')  PortDimensions=1  SampleTime=0.0001
  Select : Subsystem
  Ds : Outport  OutDataTypeStr=fixdt(1, 64, 40)  PortDimensions=1  SampleTime=0.0001  VectorParamsAs1DForOutWhenUnconnected=off
  Qs : Outport  Port=2  OutDataTypeStr=fixdt(1, 64, 40)  PortDimensions=1  SampleTime=0.0001
  wires:
  Alpha/1 -> Select/1(AlphaIn)
  Cos/1 -> Select/4(Cos)
  Beta/1 -> Select/2(BetaIn)
  Select/2(Q) -> Qs/1
  Sin/1 -> Select/3(Sin)
  Select/1(D) -> Ds/1

== system gm_PMLSM_FOC_FixedPoint/FOC_DUT/FOC_DUT/Park/Variant/mcb/sinecos ==
  note: For TI proc with fixed-point datatype
  Theta : Inport  OutDataTypeStr=fixdt(1,40,32,'DataTypeOverride', 'Off')  PortDimensions=1  SampleTime=0.0001
  Sine-Cosine Lookup : Subsystem  mask(Sine-Cosine Lookup){AngleInput=Radians, N_points=1024, DatatypeInput=Inherit from input, Datatype=Inherit: Same as input}
      mask prompts: AngleInput "shared_mcbpccmath:SinCosLib:SineBlkPrmUnits"; N_points "shared_mcbpccmath:SinCosLib:SineBlkPrmLUTSize"; DatatypeInput "shared_mcbpccmath:SinCosLib:SineBlkPrmDatatypeInput"; Datatype "shared_mcbpccmath:SinCosLib:SineBlkPrmDatatype"
      mask help: mcb:CtrlLib:SineBlkDlgDes
      mask init:
      | AngleInput = 2;
      | Datatype = 'Inherit: Same as input';
      | DatatypeInput = 1;
      | N_points = 1024;
      mask Help: eval('mcb_helpview(''sinecosinelookup'')')
      mask TypeOptions AngleInput: shared_mcbpccmath:SinCosLib:SinePopPUUnit | shared_mcbpccmath:SinCosLib:SinePopRadUnit | shared_mcbpccmath:SinCosLib:SinePopDegUnit
      mask TypeOptions DatatypeInput: shared_mcbpccmath:SinCosLib:SineBlkPopIn | shared_mcbpccmath:SinCosLib:SineBlkPopDlg
      mask Callback DatatypeInput:
      | InputFormat = get_param(gcbh,'DatatypeInput');
      | Mask = Simulink.Mask.get(gcbh);
      | Datatype = Mask.getParameter('Datatype');
      | if(strcmp(InputFormat,'Inherit from input'))
      |     Datatype.Visible = 'off';
      | else
      |     Datatype.Visible = 'on';
      | end
      mask Display: mcbpccmath.internal.drawIcons('Sin-Cos',1);
  sin : Outport  OutDataTypeStr=fixdt(1, 40, 32)  PortDimensions=1  SampleTime=0.0001
  cos : Outport  Port=2  OutDataTypeStr=fixdt(1, 40, 32)  PortDimensions=1  SampleTime=0.0001
  wires:
  Sine-Cosine Lookup/2(cos) -> cos/1
  Theta/1 -> Sine-Cosine Lookup/1(Theta)
  Sine-Cosine Lookup/1(sin) -> sin/1

== system gm_PMLSM_FOC_FixedPoint/FOC_DUT/FOC_DUT/SVPWMG/T1T2 Calculate/Fcn1/Defined_Quotient ==
  In1 : Inport
  In2 : Inport  Port=2
  Defined_Quotient : Product  Inputs=*/  OutDataTypeStr=FOC_Fixed_Config.Types.Work  RndMeth=Convergent  SaturateOnIntegerOverflow=on
  Defined_Quotient_pd1 : Delay  DelayLength=109
  Out1 : Outport
  wires:
  Defined_Quotient_pd1/1 -> Out1/1
  In1/1 -> Defined_Quotient/1
  Defined_Quotient/1 -> Defined_Quotient_pd1/1
  In2/1 -> Defined_Quotient/2

== system gm_PMLSM_FOC_FixedPoint/FOC_DUT/FOC_DUT/SVPWMG/T1T2 Calculate/Fcn2/Defined_Quotient ==
  In1 : Inport
  In2 : Inport  Port=2
  Defined_Quotient : Product  Inputs=*/  OutDataTypeStr=FOC_Fixed_Config.Types.Work  RndMeth=Convergent  SaturateOnIntegerOverflow=on
  Defined_Quotient_pd1 : Delay  DelayLength=109
  Out1 : Outport
  wires:
  Defined_Quotient_pd1/1 -> Out1/1
  In1/1 -> Defined_Quotient/1
  Defined_Quotient/1 -> Defined_Quotient_pd1/1
  In2/1 -> Defined_Quotient/2

== system gm_PMLSM_FOC_FixedPoint/FOC_DUT/FOC_DUT/InversePark/Variant/mcb/Inverse Park Transform/Select ==
  D : Inport  OutDataTypeStr=fixdt(1, 64, 40)  PortDimensions=1  SampleTime=2e-08
  Q : Inport  Port=2  OutDataTypeStr=fixdt(1, 64, 40)  PortDimensions=1  SampleTime=2e-08
  Sin : Inport  Port=3  OutDataTypeStr=fixdt(1, 40, 32)  PortDimensions=1  SampleTime=2e-08
  Cos : Inport  Port=4  OutDataTypeStr=fixdt(1, 40, 32)  PortDimensions=1  SampleTime=2e-08
  Two Inputs : Subsystem
  AlphaO : Outport  OutDataTypeStr=fixdt(1, 64, 40)  PortDimensions=1  SampleTime=2e-08  VectorParamsAs1DForOutWhenUnconnected=off
  BetaO : Outport  Port=2  OutDataTypeStr=fixdt(1, 64, 40)  PortDimensions=1  SampleTime=2e-08
  wires:
  Cos/1 -> Two Inputs/4(Cos)
  D/1 -> Two Inputs/1(D)
  Two Inputs/2(BetaO) -> BetaO/1
  Q/1 -> Two Inputs/2(Q)
  Sin/1 -> Two Inputs/3(Sin)
  Two Inputs/1(AlphaO) -> AlphaO/1
